simulink model "Chapter6"  (R2024b)
settings: Solver=ode4  StartTime=0.0  StopTime=SIM.StopTime  FixedStep=SIM.FixedStepSize  RelTol=1e-3
values from neighbouring files (symbols this model uses):
  AP = computeAutopilotGains(MAV, TRIM, TFS, DES)    [ch6_main.m]    (also in computeAutopilotGains.m = struct())
  CMD = struct()    [ch6_main.m]
  DES = loadDesignParams()    [ch6_main.m]    (also in loadDesignParams.m = struct())
  LIM = loadSafetyLimits()    [ch6_main.m]
  TRIM =     [ch6.mat]    (also in ch6_main.m = findTrim(TRIM_MODEL, Va_trim, R_trim, gamma_trim, TRIM_DATA_; findTrim.m = struct())
undefined symbols (not defined in the file or in its folder): drawAircraft, MAV, plotter, SIM
libraries: simulink x8, matrix_library x2
(part 1 of 2)
settings Model: Creator=emrec  LastModifiedBy=emrec

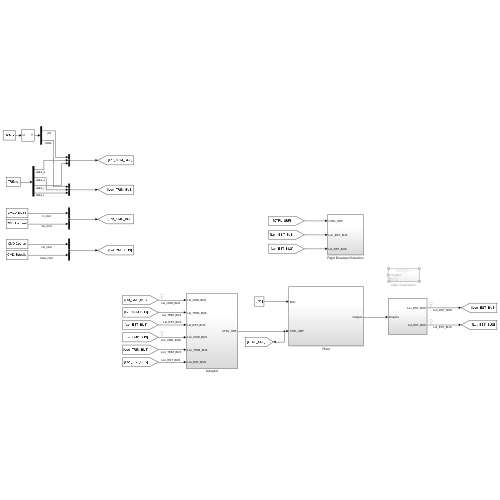
[thumbnail: Simulink's stored preview of the top-level diagram]
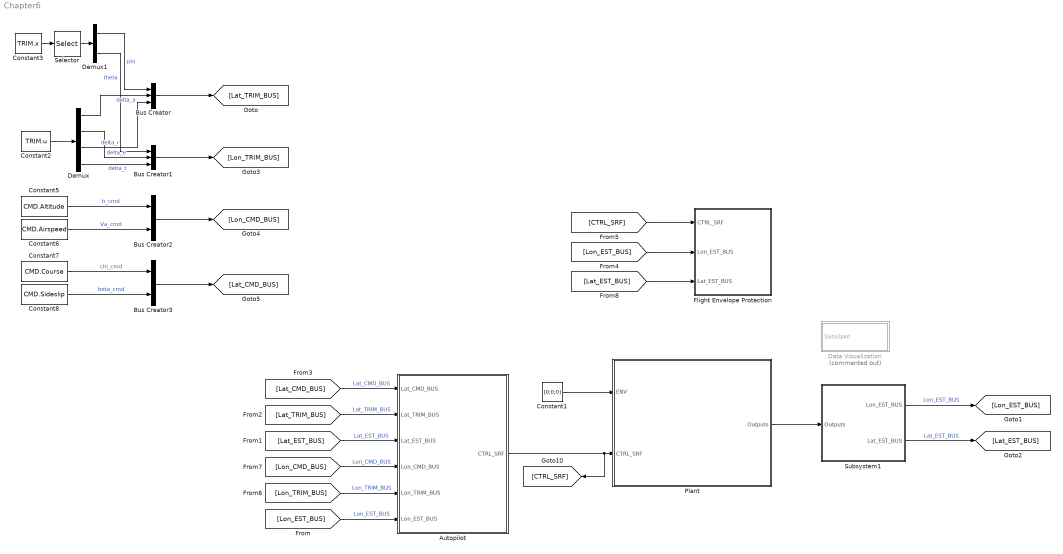
== system Chapter6 ==
  Autopilot : Subsystem
  Bus Creator : BusCreator  Inputs=3
  Bus Creator1 : BusCreator  Inputs=3
  Bus Creator2 : BusCreator  Inputs=2
  Bus Creator3 : BusCreator  Inputs=2
  Constant1 : Constant  Value=[0;0;0]
  Constant2 : Constant  Value=TRIM.u
  Constant3 : Constant  Value=TRIM.x
  Constant5 : Constant  Value=CMD.Altitude
  Constant6 : Constant  Value=CMD.Airspeed
  Constant7 : Constant  Value=CMD.Course
  Constant8 : Constant  Value=CMD.Sideslip
  Data Visualization : Subsystem  Commented=on  Variant=on
  Demux : Demux
  Demux1 : Demux  Outputs=2
  Flight Envelope Protection : Subsystem
  Plant : Subsystem
  Selector : Selector  InputPortWidth=12  IndexOptions=Index vector (dialog)  Indices=[7,8]  OutputSizes=1
  Subsystem1 : Subsystem
  wires:
  Constant1/1 -> Plant/1(ENV)
  Constant2/1 -> Demux/1
  Demux/1 -> Bus Creator/2  "delta_a"
  Demux/2 -> Bus Creator1/2  "delta_e"
  Demux/3 -> Bus Creator/3  "delta_r"
  Demux/4 -> Bus Creator1/3  "delta_t"
  Plant/1(Outputs) -> Subsystem1/1(Outputs)
  Subsystem1/1(Lon_EST_BUS) -> [Lon_EST_BUS]  "Lon_EST_BUS"
  Subsystem1/2(Lat_EST_BUS) -> [Lat_EST_BUS]  "Lat_EST_BUS"
  Bus Creator/1 -> [Lat_TRIM_BUS]
  Bus Creator1/1 -> [Lon_TRIM_BUS]
  Constant6/1 -> Bus Creator2/2  "Va_cmd"
  Constant5/1 -> Bus Creator2/1  "h_cmd"
  Bus Creator2/1 -> [Lon_CMD_BUS]
  Bus Creator3/1 -> [Lat_CMD_BUS]
  Constant7/1 -> Bus Creator3/1  "chi_cmd"
  Constant8/1 -> Bus Creator3/2  "beta_cmd"
  Constant3/1 -> Selector/1
  Selector/1 -> Demux1/1
  Demux1/1 -> Bus Creator/1  "phi"
  Demux1/2 -> Bus Creator1/1  "theta"
  Autopilot/1(CTRL_SRF) -> [CTRL_SRF], Plant/2(CTRL_SRF)
  [Lat_CMD_BUS] -> Autopilot/1(Lat_CMD_BUS)  "Lat_CMD_BUS"
  [Lat_TRIM_BUS] -> Autopilot/2(Lat_TRIM_BUS)  "Lat_TRIM_BUS"
  [Lat_EST_BUS] -> Autopilot/3(Lat_EST_BUS)  "Lat_EST_BUS"
  [Lon_CMD_BUS] -> Autopilot/4(Lon_CMD_BUS)  "Lon_CMD_BUS"
  [Lon_TRIM_BUS] -> Autopilot/5(Lon_TRIM_BUS)  "Lon_TRIM_BUS"
  [Lon_EST_BUS] -> Autopilot/6(Lon_EST_BUS)  "Lon_EST_BUS"
  [CTRL_SRF] -> Flight Envelope Protection/1(CTRL_SRF)
  [Lon_EST_BUS] -> Flight Envelope Protection/2(Lon_EST_BUS)
  [Lat_EST_BUS] -> Flight Envelope Protection/3(Lat_EST_BUS)

== system Chapter6/Autopilot ==
  Lat_CMD_BUS : Inport
  Lat_TRIM_BUS : Inport  Port=2
  Lat_EST_BUS : Inport  Port=3
  Lon_CMD_BUS : Inport  Port=4
  Lon_TRIM_BUS : Inport  Port=5
  Lon_EST_BUS : Inport  Port=6
  Lateral Autopilot : Subsystem
  Longitudinal Autopilot : Subsystem
  Mux1 : Mux
  CTRL_SRF : Outport
  wires:
  [delta_a] -> Mux1/1
  Lateral Autopilot/2(delta_r) -> [delta_r]
  [delta_t] -> Mux1/4
  Mux1/1 -> CTRL_SRF/1  "CTRL_SRF"
  Longitudinal Autopilot/1(delta_e) -> [delta_e]
  Longitudinal Autopilot/2(delta_t) -> [delta_t]
  [delta_e] -> Mux1/2
  Lon_CMD_BUS/1 -> Longitudinal Autopilot/1(Lon_CMD_BUS)
  [delta_r] -> Mux1/3
  Lateral Autopilot/1(delta_a) -> [delta_a]
  Lat_EST_BUS/1 -> Lateral Autopilot/3(Lat_EST_BUS)
  Lon_EST_BUS/1 -> Longitudinal Autopilot/3(Lon_EST_BUS)
  Lat_CMD_BUS/1 -> Lateral Autopilot/1(Lat_CMD_BUS)
  Lon_TRIM_BUS/1 -> Longitudinal Autopilot/2(Lon_TRIM_BUS)
  Lat_TRIM_BUS/1 -> Lateral Autopilot/2(Lat_TRIM_BUS)

== system Chapter6/Data Visualization ==
  note: 1) Add Subsystem or Model blocks as valid variant choices.
      | 2) You cannot connect blocks at this level. At simulation, connectivity is automatically
      | determined, based on the active variant and port name matching.
  Data2plot : Inport
  Data Storing : Subsystem  VariantControl=PLOTTING_MODEL == 2
  Online Plotting : Subsystem  VariantControl=PLOTTING_MODEL == 1

== system Chapter6/Flight Envelope Protection ==
  CTRL_SRF : Inport
  Lon_EST_BUS : Inport  Port=2
  Lat_EST_BUS : Inport  Port=3
  Abs : Abs  SaturateOnIntegerOverflow=off
  Bus Selector : BusSelector  OutputSignals=p_nh_hat,Va_hat,theta_hat
  Compare To Constant : simulink/Logic and Bit Operations/Compare To Constant  relop=<  const=LIM.Altitude.min  OutDataTypeStr=boolean
  Compare To Constant1 : simulink/Logic and Bit Operations/Compare To Constant  relop=>  const=LIM.Altitude.max  OutDataTypeStr=boolean
  Compare To Constant2 : simulink/Logic and Bit Operations/Compare To Constant  relop=>  const=LIM.Airspeed.max  OutDataTypeStr=boolean
  Compare To Constant3 : simulink/Logic and Bit Operations/Compare To Constant  relop=>  const=LIM.Pitch.max  OutDataTypeStr=boolean
  Logical Operator : Logic  Operator=OR  Inputs=4  AllPortsSameDT=off  OutDataTypeStr=boolean
  Selector : Selector  InputPortWidth=2  IndexOptions=Index vector (dialog)  Indices=[2]  OutputSizes=1
  Stop Simulation : Stop
  wires:
  Lon_EST_BUS/1 -> Bus Selector/1
  Bus Selector/1 -> Selector/1  "<p_nh_hat>"
  Selector/1 -> Compare To Constant/1, Compare To Constant1/1
  Compare To Constant/1 -> Logical Operator/1  "crash"
  Compare To Constant1/1 -> Logical Operator/2  "excess_h"
  Compare To Constant2/1 -> Logical Operator/3  "excess_Va"
  Bus Selector/3 -> Abs/1  "<theta_hat>"
  Abs/1 -> Compare To Constant3/1
  Bus Selector/2 -> Compare To Constant2/1  "<Va_hat>"
  Compare To Constant3/1 -> Logical Operator/4  "excess_theta"
  Logical Operator/1 -> Stop Simulation/1

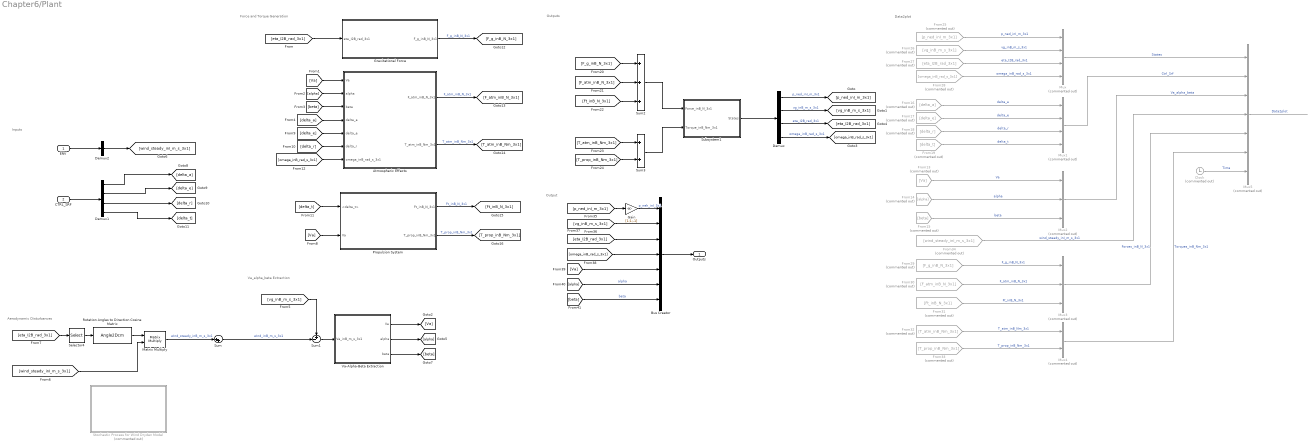
== system Chapter6/Plant ==
  note: Aerodynamic Disturbances
  note: Force and Torque Generation
  note: Inputs
  note: Outputs
  note: Data2plot
  note: Va_alpha_beta Extraction
  note: Output
  ENV : Inport
  CTRL_SRF : Inport  Port=2
  Atmospheric Effects : Subsystem
  Bus Creator : BusCreator  Inputs=7
  Clock : Clock  Commented=on
  Demux : Demux
  Demux1 : Demux
  Demux2 : Demux  Outputs=1
  From13 : From  Commented=on  GotoTag=Va
  From14 : From  Commented=on  GotoTag=alpha
  From15 : From  Commented=on  GotoTag=beta
  From16 : From  Commented=on  GotoTag=delta_a
  From17 : From  Commented=on  GotoTag=delta_e
  From18 : From  Commented=on  GotoTag=delta_r
  From19 : From  Commented=on  GotoTag=delta_t
  From25 : From  Commented=on  GotoTag=p_ned_inI_m_3x1
  From26 : From  Commented=on  GotoTag=vg_inB_m_s_3x1
  From27 : From  Commented=on  GotoTag=eta_I2B_rad_3x1
  From28 : From  Commented=on  GotoTag=omega_inB_rad_s_3x1
  From29 : From  Commented=on  GotoTag=F_g_inB_N_3x1
  From30 : From  Commented=on  GotoTag=F_atm_inB_N_3x1
  From31 : From  Commented=on  GotoTag=Ft_inB_N_3x1
  From32 : From  Commented=on  GotoTag=T_atm_inB_Nm_3x1
  From33 : From  Commented=on  GotoTag=T_prop_inB_Nm_3x1
  From34 : From  Commented=on  GotoTag=wind_steady_inI_m_s_3x1
  Gain : Gain  Gain=[1;1;-1]
  Gravitational Force : Subsystem
  Matrix Multiply : Product  Multiplication=Matrix(*)
  Mux : Mux  Commented=on
  Mux1 : Mux  Commented=on
  Mux2 : Mux  Commented=on  Inputs=3
  Mux3 : Mux  Commented=on  Inputs=3
  Mux4 : Mux  Commented=on  Inputs=2
  Mux5 : Mux  Commented=on  Inputs=7
  Propulsion System : Subsystem
  Rotation Angles to Direction Cosine Matrix : Angle2Dcm
      settings: AttributesFormatString=Rotation Order: %<rotationOrder>
  Selector4 : Selector  InputPortWidth=3  IndexOptions=Index vector (dialog)  Indices=[3 2 1]  OutputSizes=1
  Stochastic Process for Wind Dryden Model : Subsystem  Commented=on
  Subsystem1 : Subsystem  mask{init_states=MAV.init_states, J_B_B=MAV.J_B_B, m=MAV.m}
      mask prompts: init_states "Initial state values"; J_B_B "Inertia matrix (Kg.m3)"; m "Mass (Kg)"
  Sum : Sum  Inputs=|++
  Sum1 : Sum  Inputs=+-|
  Sum2 : Sum  Inputs=+++
  Sum3 : Sum
  Va-Alpha-Beta Extraction : Subsystem
  Outputs : Outport
  wires:
  Bus Creator/1 -> Outputs/1
  [omega_inB_rad_s_3x1] -> Bus Creator/4
  [eta_I2B_rad_3x1] -> Bus Creator/3
  [vg_inB_m_s_3x1] -> Bus Creator/2
  [p_ned_inI_m_3x1] -> Gain/1
  [Va] -> Propulsion System/2(Va)
  [delta_t] -> Propulsion System/1(<delta_t>)
  Propulsion System/1(Ft_inB_N_3x1) -> [Ft_inB_N_3x1]  "Ft_inB_N_3x1"
  Propulsion System/2(T_prop_inB_Nm_3x1) -> [T_prop_inB_Nm_3x1]  "T_prop_inB_Nm_3x1"
  Mux4/1 -> Mux5/6  "Torques_inB_Nm_3x1"
  Mux2/1 -> Mux5/3  "Va_alpha_beta"
  From34/1 -> Mux5/4  "wind_steady_inI_m_s_3x1"
  Clock/1 -> Mux5/7  "Time"
  Mux5/1 -> ?  "Data2plot"
  From33/1 -> Mux4/2  "T_prop_inB_Nm_3x1"
  From32/1 -> Mux4/1  "T_atm_inB_Nm_3x1"
  Mux3/1 -> Mux5/5  "Forces_inB_N_3x1"
  From29/1 -> Mux3/1  "F_g_inB_N_3x1"
  From30/1 -> Mux3/2  "F_atm_inB_N_3x1"
  From31/1 -> Mux3/3  "Ft_inB_N_3x1"
  From15/1 -> Mux2/3  "beta"
  From13/1 -> Mux2/1  "Va"
  From14/1 -> Mux2/2  "alpha"
  Mux1/1 -> Mux5/2  "Ctrl_Srf"
  From19/1 -> Mux1/4  "delta_t"
  From18/1 -> Mux1/3  "delta_r"
  From17/1 -> Mux1/2  "delta_e"
  From16/1 -> Mux1/1  "delta_a"
  Mux/1 -> Mux5/1  "States"
  From28/1 -> Mux/4  "omega_inB_rad_s_3x1"
  From27/1 -> Mux/3  "eta_I2B_rad_3x1"
  From26/1 -> Mux/2  "vg_inB_m_s_3x1"
  From25/1 -> Mux/1  "p_ned_inI_m_3x1"
  [T_prop_inB_Nm_3x1] -> Sum3/2
  [T_atm_inB_Nm_3x1] -> Sum3/1
  [Ft_inB_N_3x1] -> Sum2/3
  [F_atm_inB_N_3x1] -> Sum2/2
  [F_g_inB_N_3x1] -> Sum2/1
  Gravitational Force/1(F_g_inB_N_3x1) -> [F_g_inB_N_3x1]  "F_g_inB_N_3x1"
  Atmospheric Effects/1(F_atm_inB_N_3x1) -> [F_atm_inB_N_3x1]  "F_atm_inB_N_3x1"
  Atmospheric Effects/2(T_atm_inB_Nm_3x1) -> [T_atm_inB_Nm_3x1]  "T_atm_inB_Nm_3x1"
  Demux1/2 -> [delta_e]
  ENV/1 -> Demux2/1
  Sum1/1 -> Va-Alpha-Beta Extraction/1(Va_inB_m_s_3x1)
  [wind_steady_inI_m_s_3x1] -> Matrix Multiply/2
  Demux2/1 -> [wind_steady_inI_m_s_3x1]
  Selector4/1 -> Rotation Angles to Direction Cosine Matrix/1
  Demux1/4 -> [delta_t]
  [Va] -> Atmospheric Effects/1(Va)
  Va-Alpha-Beta Extraction/1(Va) -> [Va]
  Demux/4 -> [omega_inB_rad_s_3x1]  "omega_inB_rad_s_3x1"
  [delta_r] -> Atmospheric Effects/6(delta_r)
  [delta_a] -> Atmospheric Effects/4(delta_a)
  Matrix Multiply/1 -> Sum/1  "wind_steady_inB_m_s_3x1"
  [delta_e] -> Atmospheric Effects/5(delta_e)
  Subsystem1/1(States) -> Demux/1
  Va-Alpha-Beta Extraction/3(beta) -> [beta]
  Demux/1 -> [p_ned_inI_m_3x1]  "p_ned_inI_m_3x1"
  CTRL_SRF/1 -> Demux1/1
  Demux1/1 -> [delta_a]
  Demux/3 -> [eta_I2B_rad_3x1]  "eta_I2B_rad_3x1"
  Sum/1 -> Sum1/2  "wind_inB_m_s_3x1"
  [vg_inB_m_s_3x1] -> Sum1/1
  Demux/2 -> [vg_inB_m_s_3x1]  "vg_inB_m_s_3x1"
  [eta_I2B_rad_3x1] -> Selector4/1
  Rotation Angles to Direction Cosine Matrix/1 -> Matrix Multiply/1
  [eta_I2B_rad_3x1] -> Gravitational Force/1(eta_I2B_rad_3x1)
  Sum3/1 -> Subsystem1/2(Torque_inB_Nm_3x1)
  Va-Alpha-Beta Extraction/2(alpha) -> [alpha]
  Sum2/1 -> Subsystem1/1(Force_inB_N_3x1)
  [alpha] -> Atmospheric Effects/2(alpha)
  [beta] -> Atmospheric Effects/3(beta)
  Demux1/3 -> [delta_r]
  [omega_inB_rad_s_3x1] -> Atmospheric Effects/7(omega_inB_rad_s_3x1)
  [Va] -> Bus Creator/5
  [alpha] -> Bus Creator/6  "alpha"
  [beta] -> Bus Creator/7  "beta"
  Gain/1 -> Bus Creator/1  "p_neh_inI_3x1"

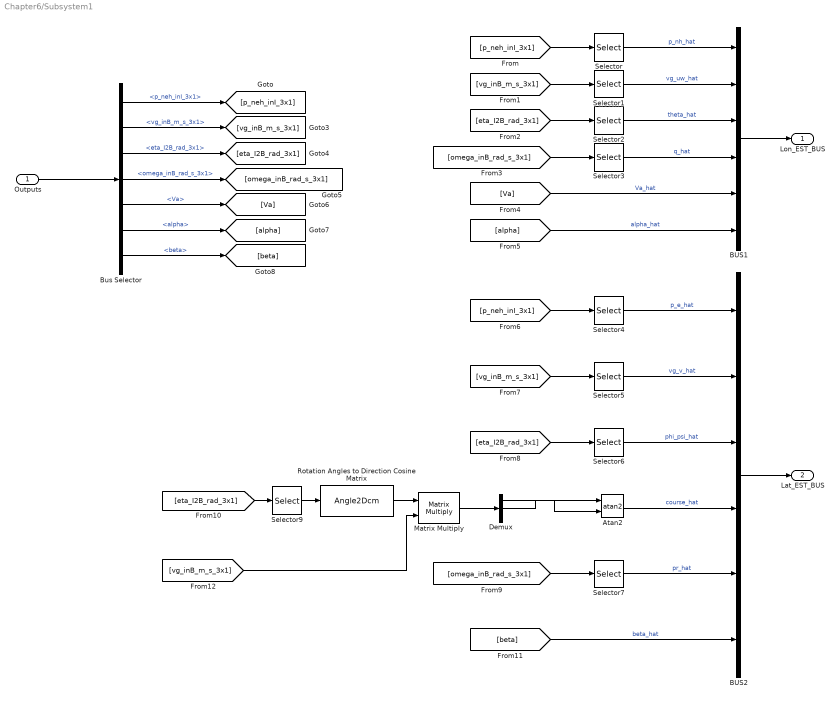
== system Chapter6/Subsystem1 ==
  Outputs : Inport
  Atan2 : Trigonometry  Operator=atan2
  BUS1 : BusCreator  Inputs=6
  BUS2 : BusCreator  Inputs=6
  Bus Selector : BusSelector  OutputSignals=p_neh_inI_3x1,vg_inB_m_s_3x1,eta_I2B_rad_3x1,omega_inB_rad_s_3x1,Va,alpha,beta
  Demux : Demux  Outputs=3
  Matrix Multiply : Product  Multiplication=Matrix(*)
  Rotation Angles to Direction Cosine Matrix : Angle2Dcm
      settings: AttributesFormatString=Rotation Order: %<rotationOrder>
  Selector : Selector  InputPortWidth=3  IndexOptions=Index vector (dialog)  Indices=[1 3]  OutputSizes=1
  Selector1 : Selector  InputPortWidth=3  IndexOptions=Index vector (dialog)  Indices=[1 3]  OutputSizes=1
  Selector{2..5} (4 alike) : Selector  InputPortWidth=3  IndexOptions=Index vector (dialog)  Indices=[2]  OutputSizes=1
  Selector6 : Selector  InputPortWidth=3  IndexOptions=Index vector (dialog)  Indices=[1,3]  OutputSizes=1
  Selector7 : Selector  InputPortWidth=3  IndexOptions=Index vector (dialog)  Indices=[1, 3]  OutputSizes=1
  Selector9 : Selector  InputPortWidth=3  IndexOptions=Index vector (dialog)  Indices=[3 2 1]  OutputSizes=1
  Lon_EST_BUS : Outport
  Lat_EST_BUS : Outport  Port=2
  wires:
  Outputs/1 -> Bus Selector/1
  BUS1/1 -> Lon_EST_BUS/1
  Bus Selector/1 -> [p_neh_inI_3x1]  "<p_neh_inI_3x1>"
  Bus Selector/2 -> [vg_inB_m_s_3x1]  "<vg_inB_m_s_3x1>"
  Bus Selector/3 -> [eta_I2B_rad_3x1]  "<eta_I2B_rad_3x1>"
  Bus Selector/4 -> [omega_inB_rad_s_3x1]  "<omega_inB_rad_s_3x1>"
  Bus Selector/5 -> [Va]  "<Va>"
  Bus Selector/6 -> [alpha]  "<alpha>"
  Bus Selector/7 -> [beta]  "<beta>"
  [p_neh_inI_3x1] -> Selector/1
  Selector/1 -> BUS1/1  "p_nh_hat"
  [vg_inB_m_s_3x1] -> Selector1/1
  Selector1/1 -> BUS1/2  "vg_uw_hat"
  [eta_I2B_rad_3x1] -> Selector2/1
  Selector2/1 -> BUS1/3  "theta_hat"
  [omega_inB_rad_s_3x1] -> Selector3/1
  Selector3/1 -> BUS1/4  "q_hat"
  [Va] -> BUS1/5  "Va_hat"
  [alpha] -> BUS1/6  "alpha_hat"
  [beta] -> BUS2/6  "beta_hat"
  Selector7/1 -> BUS2/5  "pr_hat"
  [omega_inB_rad_s_3x1] -> Selector7/1
  Selector6/1 -> BUS2/3  "phi_psi_hat"
  [eta_I2B_rad_3x1] -> Selector6/1
  Selector5/1 -> BUS2/2  "vg_v_hat"
  [vg_inB_m_s_3x1] -> Selector5/1
  Selector4/1 -> BUS2/1  "p_e_hat"
  [p_neh_inI_3x1] -> Selector4/1
  BUS2/1 -> Lat_EST_BUS/1
  Atan2/1 -> BUS2/4  "course_hat"
  [vg_inB_m_s_3x1] -> Matrix Multiply/2
  Selector9/1 -> Rotation Angles to Direction Cosine Matrix/1
  Rotation Angles to Direction Cosine Matrix/1 -> Matrix Multiply/1
  [eta_I2B_rad_3x1] -> Selector9/1
  Matrix Multiply/1 -> Demux/1
  Demux/2 -> Atan2/1
  Demux/1 -> Atan2/2

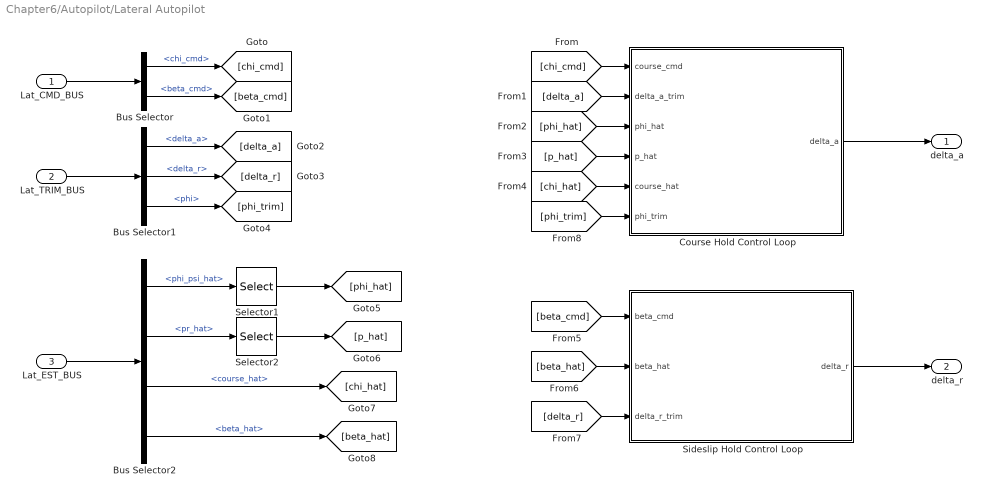
== system Chapter6/Autopilot/Lateral Autopilot ==
  Lat_CMD_BUS : Inport
  Lat_TRIM_BUS : Inport  Port=2
  Lat_EST_BUS : Inport  Port=3
  Bus Selector : BusSelector  OutputSignals=chi_cmd,beta_cmd
  Bus Selector1 : BusSelector  OutputSignals=delta_a,delta_r,phi
  Bus Selector2 : BusSelector  OutputSignals=phi_psi_hat,pr_hat,course_hat,beta_hat
  Course Hold Control Loop : Subsystem
  Selector1 : Selector  InputPortWidth=2  IndexOptions=Index vector (dialog)  Indices=1  OutputSizes=1
  Selector2 : Selector  InputPortWidth=2  IndexOptions=Index vector (dialog)  Indices=1  OutputSizes=1
  Sideslip Hold Control Loop : Subsystem
  delta_a : Outport
  delta_r : Outport  Port=2
  wires:
  Sideslip Hold Control Loop/1(delta_r) -> delta_r/1
  Course Hold Control Loop/1(delta_a) -> delta_a/1
  Lat_CMD_BUS/1 -> Bus Selector/1
  Bus Selector/1 -> [chi_cmd]  "<chi_cmd>"
  Bus Selector/2 -> [beta_cmd]  "<beta_cmd>"
  Lat_TRIM_BUS/1 -> Bus Selector1/1
  Bus Selector1/1 -> [delta_a]  "<delta_a>"
  Bus Selector1/2 -> [delta_r]  "<delta_r>"
  Lat_EST_BUS/1 -> Bus Selector2/1
  Selector1/1 -> [phi_hat]
  Bus Selector2/2 -> Selector2/1  "<pr_hat>"
  Bus Selector2/1 -> Selector1/1  "<phi_psi_hat>"
  Selector2/1 -> [p_hat]
  Bus Selector2/3 -> [chi_hat]  "<course_hat>"
  Bus Selector2/4 -> [beta_hat]  "<beta_hat>"
  [chi_cmd] -> Course Hold Control Loop/1(course_cmd)
  [delta_a] -> Course Hold Control Loop/2(delta_a_trim)
  [phi_hat] -> Course Hold Control Loop/3(phi_hat)
  [p_hat] -> Course Hold Control Loop/4(p_hat)
  [chi_hat] -> Course Hold Control Loop/5(course_hat)
  [beta_cmd] -> Sideslip Hold Control Loop/1(beta_cmd)
  [beta_hat] -> Sideslip Hold Control Loop/2(beta_hat)
  [delta_r] -> Sideslip Hold Control Loop/3(delta_r_trim)
  Bus Selector1/3 -> [phi_trim]  "<phi>"
  [phi_trim] -> Course Hold Control Loop/6(phi_trim)

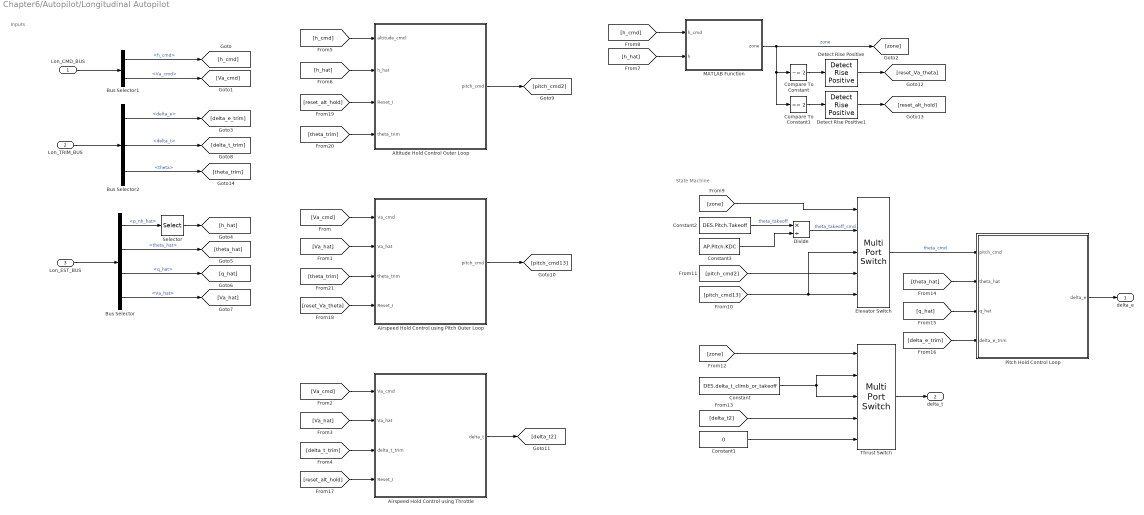
== system Chapter6/Autopilot/Longitudinal Autopilot ==
  note: Inputs
  note: State Machine
  Lon_CMD_BUS : Inport
  Lon_TRIM_BUS : Inport  Port=2
  Lon_EST_BUS : Inport  Port=3
  Airspeed Hold Control using Pitch Outer Loop : Subsystem
  "Airspeed Hold Control using Throttle " : Subsystem
  Altitude Hold Control Outer Loop : Subsystem
  Bus Selector : BusSelector  OutputSignals=p_nh_hat,theta_hat,q_hat,Va_hat
  Bus Selector1 : BusSelector  OutputSignals=h_cmd,Va_cmd
  Bus Selector2 : BusSelector  OutputSignals=delta_e,delta_t,theta
  Compare To Constant : simulink/Logic and Bit Operations/Compare To Constant  relop=~=  const=2  OutDataTypeStr=boolean
  Compare To Constant1 : simulink/Logic and Bit Operations/Compare To Constant  relop===  const=2  OutDataTypeStr=boolean
  Constant : Constant  Value=DES.delta_t_climb_or_takeoff
  Constant1 : Constant  Value=0
  Constant2 : Constant  Value=DES.Pitch.Takeoff
  Constant3 : Constant  Value=AP.Pitch.KDC
  Detect Rise Positive : simulink/Logic and Bit Operations/Detect Rise Positive  vinit=0  OutDataTypeStr=boolean
  Detect Rise Positive1 : simulink/Logic and Bit Operations/Detect Rise Positive  vinit=0  OutDataTypeStr=boolean
  Divide : Product  Inputs=*/
  Elevator Switch : MultiPortSwitch  DataPortOrder=Zero-based contiguous  Inputs=4  zeroidx=on  SaturateOnIntegerOverflow=off  InputSameDT=off
  MATLAB Function : MATLAB Function  TreatAsAtomicUnit=on  SystemSampleTime=SIM.FixedStepSize
  Pitch Hold Control Loop : Subsystem
  Selector : Selector  InputPortWidth=2  IndexOptions=Index vector (dialog)  Indices=2  OutputSizes=1
  Thrust Switch : MultiPortSwitch  DataPortOrder=Zero-based contiguous  Inputs=4  zeroidx=on  SaturateOnIntegerOverflow=off  InputSameDT=off
  delta_e : Outport
  delta_t : Outport  Port=2
  wires:
  Pitch Hold Control Loop/1(delta_e) -> delta_e/1
  [h_hat] -> MATLAB Function/2(h)
  Constant/1 -> Thrust Switch/2, Thrust Switch/3
  Constant1/1 -> Thrust Switch/5
  Thrust Switch/1 -> delta_t/1
  Constant2/1 -> Divide/1  "theta_takeoff"
  Constant3/1 -> Divide/2
  Divide/1 -> Elevator Switch/2  "theta_takeoff_cmd"
  [Va_cmd] -> Airspeed Hold Control using Pitch Outer Loop/1(Va_cmd)
  [Va_hat] -> Airspeed Hold Control using Pitch Outer Loop/2(Va_hat)
  Lon_EST_BUS/1 -> Bus Selector/1
  Bus Selector/1 -> Selector/1  "<p_nh_hat>"
  Selector/1 -> [h_hat]
  Bus Selector/2 -> [theta_hat]  "<theta_hat>"
  Bus Selector/3 -> [q_hat]  "<q_hat>"
  Bus Selector/4 -> [Va_hat]  "<Va_hat>"
  Lon_CMD_BUS/1 -> Bus Selector1/1
  Bus Selector1/1 -> [h_cmd]  "<h_cmd>"
  Bus Selector1/2 -> [Va_cmd]  "<Va_cmd>"
  Bus Selector2/1 -> [delta_e_trim]  "<delta_e>"
  Lon_TRIM_BUS/1 -> Bus Selector2/1
  Bus Selector2/2 -> [delta_t_trim]  "<delta_t>"
  [Va_cmd] -> "Airspeed Hold Control using Throttle "/1(Va_cmd)
  [Va_hat] -> "Airspeed Hold Control using Throttle "/2(Va_hat)
  [delta_t_trim] -> "Airspeed Hold Control using Throttle "/3(delta_t_trim)
  [h_cmd] -> Altitude Hold Control Outer Loop/1(altitude_cmd)
  [h_hat] -> Altitude Hold Control Outer Loop/2(h_hat)
  Altitude Hold Control Outer Loop/1(pitch_cmd) -> [pitch_cmd2]
  Airspeed Hold Control using Pitch Outer Loop/1(pitch_cmd) -> [pitch_cmd13]
  "Airspeed Hold Control using Throttle "/1(delta_t) -> [delta_t2]
  [h_cmd] -> MATLAB Function/1(h_cmd)
  [zone] -> Elevator Switch/1
  [pitch_cmd13] -> Elevator Switch/5, Elevator Switch/3
  [pitch_cmd2] -> Elevator Switch/4
  [zone] -> Thrust Switch/1
  [delta_t2] -> Thrust Switch/4
  [theta_hat] -> Pitch Hold Control Loop/2(theta_hat)
  [q_hat] -> Pitch Hold Control Loop/3(q_hat)
  [delta_e_trim] -> Pitch Hold Control Loop/4(delta_e_trim)
  Compare To Constant/1 -> Detect Rise Positive/1
  Compare To Constant1/1 -> Detect Rise Positive1/1
  Detect Rise Positive/1 -> [reset_Va_theta]
  Detect Rise Positive1/1 -> [reset_alt_hold]
  [reset_alt_hold] -> "Airspeed Hold Control using Throttle "/4(Reset_I)
  [reset_Va_theta] -> Airspeed Hold Control using Pitch Outer Loop/4(Reset_I)
  [reset_alt_hold] -> Altitude Hold Control Outer Loop/3(Reset_I)
  Bus Selector2/3 -> [theta_trim]  "<theta>"
  [theta_trim] -> Altitude Hold Control Outer Loop/4(theta_trim)
  [theta_trim] -> Airspeed Hold Control using Pitch Outer Loop/3(theta_trim)
  MATLAB Function/1(zone) -> [zone], Compare To Constant1/1, Compare To Constant/1  "zone"
  Elevator Switch/1 -> Pitch Hold Control Loop/1(pitch_cmd)  "theta_cmd"

== system Chapter6/Data Visualization/Data Storing ==
  Data2plot : Inport
  To Workspace : ToWorkspace  VariableName=simout  SampleTime=-1
  wires:
  Data2plot/1 -> To Workspace/1

== system Chapter6/Data Visualization/Online Plotting ==
  Data2plot : Inport
  Aircraft Body Animation : MATLABFcn  MATLABFcn=drawAircraft(u)  OutputDimensions=0
  Clock : Clock
  Mux : Mux  Inputs=2
  Plot Graphs : MATLABFcn  MATLABFcn=plotter(u)  OutputDimensions=0
  Selector : Selector  InputPortWidth=38  IndexOptions=Index vector (dialog)  Indices=[1:12]  OutputSizes=1
  wires:
  Mux/1 -> Aircraft Body Animation/1
  Clock/1 -> Mux/2
  Selector/1 -> Mux/1
  Data2plot/1 -> Plot Graphs/1, Selector/1

== system Chapter6/Plant/Atmospheric Effects ==
  Va : Inport
  alpha : Inport  Port=2
  beta : Inport  Port=3
  delta_a : Inport  Port=4
  delta_e : Inport  Port=5
  delta_r : Inport  Port=6
  omega_inB_rad_s_3x1 : Inport  Port=7
  Aerodynamic Effect on Latitude Motion : Subsystem
  Aerodynamic Effect on Longitudinal Motion : Subsystem
  Mux1 : Mux  Inputs=2
  Selector : Selector  InputPortWidth=3  IndexOptions=Index vector (dialog)  Indices=[2]  OutputSizes=1
  Selector1 : Selector  InputPortWidth=3  IndexOptions=Index vector (dialog)  Indices=[1 3]  OutputSizes=1
  Selector2 : Selector  InputPortWidth=6  IndexOptions=Index vector (dialog)  Indices=[1 4 2]  OutputSizes=1
  Selector3 : Selector  InputPortWidth=6  IndexOptions=Index vector (dialog)  Indices=[5 3 6]  OutputSizes=1
  F_atm_inB_N_3x1 : Outport
  T_atm_inB_Nm_3x1 : Outport  Port=2
  wires:
  Mux1/1 -> Selector3/1, Selector2/1
  Selector2/1 -> F_atm_inB_N_3x1/1  "F_atm_inB_N_3x1"
  delta_e/1 -> Aerodynamic Effect on Longitudinal Motion/1(delta_e)
  delta_a/1 -> Aerodynamic Effect on Latitude Motion/1(delta_a)
  Aerodynamic Effect on Longitudinal Motion/1(Fx_Fz_Tq_inB) -> Mux1/1
  alpha/1 -> Aerodynamic Effect on Longitudinal Motion/3(alpha)
  Aerodynamic Effect on Latitude Motion/1(Fy_Tp_Tr_inB) -> Mux1/2
  delta_r/1 -> Aerodynamic Effect on Latitude Motion/2(delta_r)
  omega_inB_rad_s_3x1/1 -> Selector1/1, Selector/1
  Va/1 -> Aerodynamic Effect on Latitude Motion/5(Va), Aerodynamic Effect on Longitudinal Motion/4(Va)
  beta/1 -> Aerodynamic Effect on Latitude Motion/3(beta)
  Selector3/1 -> T_atm_inB_Nm_3x1/1  "T_atm_inB_Nm_3x1"
  Selector/1 -> Aerodynamic Effect on Longitudinal Motion/2(q)
  Selector1/1 -> Aerodynamic Effect on Latitude Motion/4(p_r)

== system Chapter6/Plant/Gravitational Force ==
  eta_I2B_rad_3x1 : Inport
  Constant : Constant  Value=MAV.m * MAV.g
  Product : Product
  R_B_I_c3 : MATLAB Function  TreatAsAtomicUnit=on
  F_g_inB_N_3x1 : Outport
  wires:
  eta_I2B_rad_3x1/1 -> R_B_I_c3/1(u)
  R_B_I_c3/1(y) -> Product/1
  Constant/1 -> Product/2  "F_g_inI_N_3x1"
  Product/1 -> F_g_inB_N_3x1/1  "F_g_inB_N_3x1"

== system Chapter6/Plant/Propulsion System ==
  <delta_t> : Inport
  Va : Inport  Port=2
  Gain2 : Gain  Gain=MAV.K_motor
  Gain3 : Gain  Gain=MAV.S_prop * MAV.C_prop * MAV.rho/ 2
  Gain4 : Gain  Gain=-MAV.K_t_prop
  Gain5 : Gain  Gain=MAV.K_omega
  Square1 : Math  Operator=square
  Square2 : Math  Operator=square
  Square3 : Math  Operator=square
  Sum2 : Sum  Inputs=|+-
  vectorize_e1 : Gain  Gain=[1;0;0]
  vectorize_e2 : Gain  Gain=[1;0;0]
  Ft_inB_N_3x1 : Outport
  T_prop_inB_Nm_3x1 : Outport  Port=2
  wires:
  Gain5/1 -> Square3/1  "V_exit"
  Square3/1 -> Gain4/1
  vectorize_e2/1 -> T_prop_inB_Nm_3x1/1  "T_prop_inB_Nm_3x1"
  Va/1 -> Square2/1
  <delta_t>/1 -> Gain5/1, Gain2/1
  Gain3/1 -> Ft_inB_N_3x1/1  "Ft_inB_N_3x1"
  vectorize_e1/1 -> Gain3/1
  Square2/1 -> Sum2/2
  Sum2/1 -> vectorize_e1/1
  Gain4/1 -> vectorize_e2/1
  Square1/1 -> Sum2/1
  Gain2/1 -> Square1/1  "V_exit"

== system Chapter6/Plant/Stochastic Process for Wind Dryden Model ==

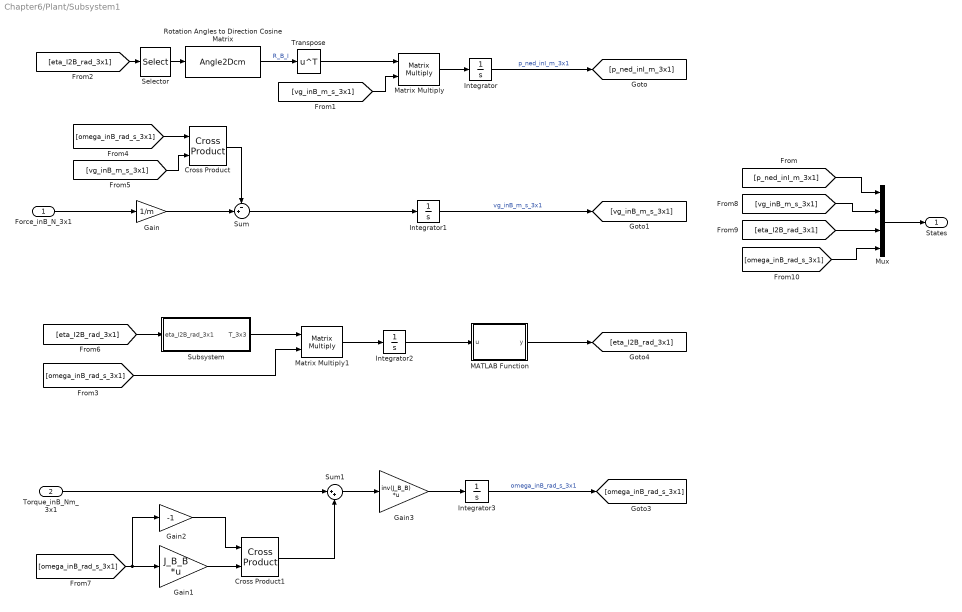
== system Chapter6/Plant/Subsystem1 ==
  Force_inB_N_3x1 : Inport
  Torque_inB_Nm_3x1 : Inport  Port=2
  Cross Product : matrix_library/Cross Product
  Cross Product1 : matrix_library/Cross Product
  Gain : Gain  Gain=1/m
  Gain1 : Gain  Gain=J_B_B  Multiplication=Matrix(K*u)
  Gain2 : Gain  Gain=-1
  Gain3 : Gain  Gain=inv(J_B_B)  Multiplication=Matrix(K*u)
  Integrator : Integrator  InitialCondition=init_states(1:3)
  Integrator1 : Integrator  InitialCondition=init_states(4:6)
  Integrator2 : Integrator  InitialCondition=init_states(7:9)
  Integrator3 : Integrator  InitialCondition=init_states(10:12)
  MATLAB Function : MATLAB Function  TreatAsAtomicUnit=on
  Matrix Multiply : Product  Multiplication=Matrix(*)
  Matrix Multiply1 : Product  Multiplication=Matrix(*)
  Mux : Mux
  Rotation Angles to Direction Cosine Matrix : Angle2Dcm
      settings: AttributesFormatString=Rotation Order: %<rotationOrder>
  Selector : Selector  InputPortWidth=3  IndexOptions=Index vector (dialog)  Indices=[3;2;1]  OutputSizes=1
  Subsystem : Subsystem
  Sum : Sum  Inputs=-+|
  Sum1 : Sum  Inputs=|++
  Transpose : Math  Operator=transpose
  States : Outport
  wires:
  MATLAB Function/1(y) -> [eta_I2B_rad_3x1]
  Gain3/1 -> Integrator3/1
  [p_ned_inI_m_3x1] -> Mux/1
  [omega_inB_rad_s_3x1] -> Cross Product/1
  Matrix Multiply1/1 -> Integrator2/1
  Gain1/1 -> Cross Product1/2
  [eta_I2B_rad_3x1] -> Subsystem/1(eta_I2B_rad_3x1)
  [omega_inB_rad_s_3x1] -> Matrix Multiply1/2
  Integrator1/1 -> [vg_inB_m_s_3x1]  "vg_inB_m_s_3x1"
  [vg_inB_m_s_3x1] -> Cross Product/2
  Selector/1 -> Rotation Angles to Direction Cosine Matrix/1
  [eta_I2B_rad_3x1] -> Selector/1
  Cross Product/1 -> Sum/1
  Integrator/1 -> [p_ned_inI_m_3x1]  "p_ned_inI_m_3x1"
  Matrix Multiply/1 -> Integrator/1
  Force_inB_N_3x1/1 -> Gain/1
  Rotation Angles to Direction Cosine Matrix/1 -> Transpose/1  "R_B_I"
  [omega_inB_rad_s_3x1] -> Gain2/1, Gain1/1
  Mux/1 -> States/1
  [omega_inB_rad_s_3x1] -> Mux/4
  Transpose/1 -> Matrix Multiply/1
  Integrator3/1 -> [omega_inB_rad_s_3x1]  "omega_inB_rad_s_3x1"
  [vg_inB_m_s_3x1] -> Matrix Multiply/2
  [eta_I2B_rad_3x1] -> Mux/3
  Torque_inB_Nm_3x1/1 -> Sum1/1
  Gain2/1 -> Cross Product1/1
  Sum1/1 -> Gain3/1
  Integrator2/1 -> MATLAB Function/1(u)
  [vg_inB_m_s_3x1] -> Mux/2
  Subsystem/1(T_3x3) -> Matrix Multiply1/1
  Cross Product1/1 -> Sum1/2
  Sum/1 -> Integrator1/1
  Gain/1 -> Sum/2

== system Chapter6/Plant/Va-Alpha-Beta Extraction ==
  note: To avoid zero division problem.
      | This logic and threshold is recommended by gemini.
  note: Va >= ||vr|| -> Va = 0 -> vr = 0
  Va_inB_m_s_3x1 : Inport
  Asin : Trigonometry  Operator=asin
  Constant : Constant
  Demux : Demux  Outputs=3
  Divide1 : Product  Inputs=*/
  Switch : Switch  Criteria=u2 > Threshold  SaturateOnIntegerOverflow=off  InputSameDT=off
  Trigonometric Function : Trigonometry  Operator=atan2  OutputSignalType=real
  norm2 : Subsystem
  Va : Outport
  alpha : Outport  Port=2
  beta : Outport  Port=3
  wires:
  Va_inB_m_s_3x1/1 -> norm2/1(Va_inB_m_s_3x1), Demux/1
  Demux/1 -> Trigonometric Function/2  "ur"
  Demux/2 -> Divide1/1  "vr"
  Demux/3 -> Trigonometric Function/1  "wr"
  norm2/1(Va) -> Switch/2, Switch/1, Va/1  "Va"
  Divide1/1 -> Asin/1
  Asin/1 -> beta/1
  Trigonometric Function/1 -> alpha/1
  Constant/1 -> Switch/3
  Switch/1 -> Divide1/2

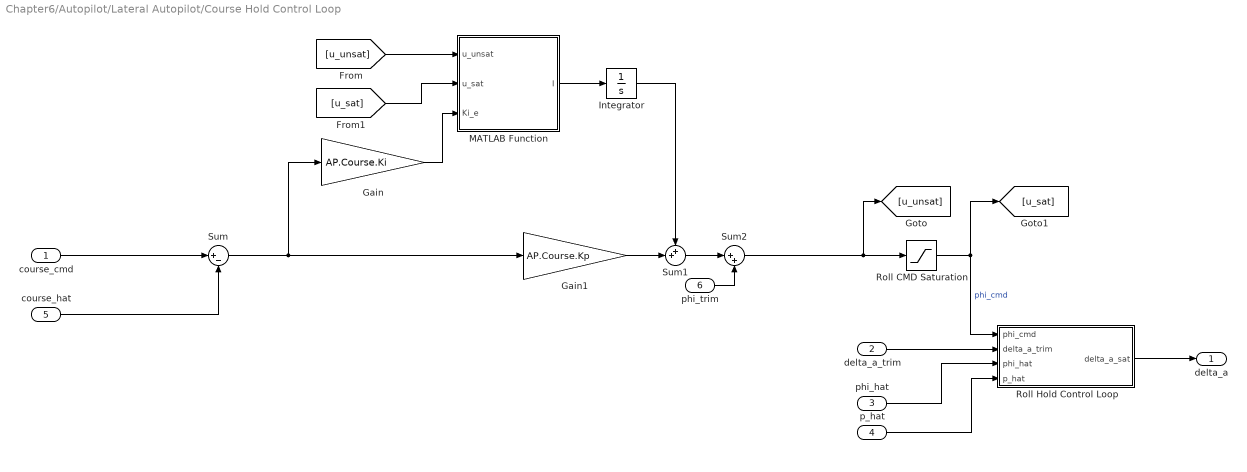
== system Chapter6/Autopilot/Lateral Autopilot/Course Hold Control Loop ==
  course_cmd : Inport
  delta_a_trim : Inport  Port=2
  phi_hat : Inport  Port=3
  p_hat : Inport  Port=4
  course_hat : Inport  Port=5
  phi_trim : Inport  Port=6
  Gain : Gain  Gain=AP.Course.Ki
  Gain1 : Gain  Gain=AP.Course.Kp
  Integrator : Integrator
  MATLAB Function : MATLAB Function  TreatAsAtomicUnit=on
  "Roll CMD Saturation " : Saturate  UpperLimit=DES.Roll.max  LowerLimit=-DES.Roll.max
  Roll Hold Control Loop : Subsystem
  Sum : Sum  Inputs=|+-
  Sum1 : Sum  Inputs=++|
  Sum2 : Sum  Inputs=|++
  delta_a : Outport
  wires:
  p_hat/1 -> Roll Hold Control Loop/4(p_hat)
  Integrator/1 -> Sum1/1
  Sum/1 -> Gain1/1, Gain/1
  Gain1/1 -> Sum1/2
  phi_hat/1 -> Roll Hold Control Loop/3(phi_hat)
  course_cmd/1 -> Sum/1
  course_hat/1 -> Sum/2
  delta_a_trim/1 -> Roll Hold Control Loop/2(delta_a_trim)
  Roll Hold Control Loop/1(delta_a_sat) -> delta_a/1
  Sum2/1 -> [u_unsat], "Roll CMD Saturation "/1
  "Roll CMD Saturation "/1 -> Roll Hold Control Loop/1(phi_cmd), [u_sat]  "phi_cmd"
  Gain/1 -> MATLAB Function/3(Ki_e)
  [u_unsat] -> MATLAB Function/1(u_unsat)
  [u_sat] -> MATLAB Function/2(u_sat)
  MATLAB Function/1(I) -> Integrator/1
  Sum1/1 -> Sum2/1
  phi_trim/1 -> Sum2/2

== system Chapter6/Autopilot/Lateral Autopilot/Sideslip Hold Control Loop ==
  beta_cmd : Inport
  beta_hat : Inport  Port=2
  delta_r_trim : Inport  Port=3
  Gain : Gain  Gain=-AP.Sideslip.Ki
  Gain1 : Gain  Gain=-AP.Sideslip.Kp
  MATLAB Function : MATLAB Function  TreatAsAtomicUnit=on
  Rudder Saturation : Saturate  UpperLimit=DES.delta_r_max  LowerLimit=-DES.delta_r_max
  Sideslip Hold I Action : Integrator
  Sum : Sum  Inputs=|+-
  Sum1 : Sum  Inputs=++|
  Sum2 : Sum  Inputs=|++
  delta_r : Outport
  wires:
  beta_cmd/1 -> Sum/1
  delta_r_trim/1 -> Sum2/2
  Sum1/1 -> Sum2/1  "Ddelta_r"
  Sum/1 -> Gain1/1, Gain/1
  Sum2/1 -> [u_unsat], Rudder Saturation/1
  Gain1/1 -> Sum1/2
  Rudder Saturation/1 -> [u_sat], delta_r/1  "delta_r_sat"
  beta_hat/1 -> Sum/2
  Sideslip Hold I Action/1 -> Sum1/1
  Gain/1 -> MATLAB Function/3(Ki_e)
  MATLAB Function/1(I) -> Sideslip Hold I Action/1
  [u_unsat] -> MATLAB Function/1(u_unsat)
  [u_sat] -> MATLAB Function/2(u_sat)

== system Chapter6/Autopilot/Longitudinal Autopilot/Airspeed Hold Control using Pitch Outer Loop ==
  Va_cmd : Inport
  Va_hat : Inport  Port=2
  theta_trim : Inport  Port=3
  Reset_I : Inport  Port=4
  Airspeed Hold using Pitch I Action : Integrator  ExternalReset=rising
  Gain1 : Gain  Gain=AP.Airspeed.Pitch.Kp
  Gain2 : Gain  Gain=AP.Airspeed.Pitch.Ki
  MATLAB Function : MATLAB Function  TreatAsAtomicUnit=on
  Pitch CMD Saturation : Saturate  UpperLimit=DES.Airspeed.Pitch.max  LowerLimit=-DES.Airspeed.Pitch.max
  Sum : Sum  Inputs=|+-
  Sum1 : Sum  Inputs=++|
  Sum2 : Sum  Inputs=|++
  pitch_cmd : Outport
  wires:
  Va_cmd/1 -> Sum/1
  Pitch CMD Saturation/1 -> pitch_cmd/1, [u_sat]  "pitch_cmd"
  Sum/1 -> Gain1/1, Gain2/1
  [u_unsat] -> MATLAB Function/1(u_unsat)
  MATLAB Function/1(I) -> Airspeed Hold using Pitch I Action/1
  [u_sat] -> MATLAB Function/2(u_sat)
  Gain1/1 -> Sum1/2
  Gain2/1 -> MATLAB Function/3(Ki_e)
  Airspeed Hold using Pitch I Action/1 -> Sum1/1
  Va_hat/1 -> Sum/2
  Reset_I/1 -> Airspeed Hold using Pitch I Action/2
  theta_trim/1 -> Sum2/2
  Sum1/1 -> Sum2/1  "Dtheta"
  Sum2/1 -> [u_unsat], Pitch CMD Saturation/1

== system Chapter6/Autopilot/Longitudinal Autopilot/Airspeed Hold Control using Throttle  ==
  Va_cmd : Inport
  Va_hat : Inport  Port=2
  delta_t_trim : Inport  Port=3
  Reset_I : Inport  Port=4
  Airspeed Hold using Throttle I Action : Integrator  ExternalReset=rising
  Gain1 : Gain  Gain=AP.Airspeed.Throttle.Kp
  Gain2 : Gain  Gain=AP.Airspeed.Throttle.Ki
  MATLAB Function : MATLAB Function  TreatAsAtomicUnit=on
  Sum : Sum  Inputs=|+-
  Sum1 : Sum  Inputs=++|
  Sum2 : Sum  Inputs=|++
  Throttle Saturation : Saturate  UpperLimit=DES.delta_t_max  LowerLimit=0
  delta_t : Outport
  wires:
  Va_hat/1 -> Sum/2
  Airspeed Hold using Throttle I Action/1 -> Sum1/1
  Gain2/1 -> MATLAB Function/3(Ki_e)
  Gain1/1 -> Sum1/2
  [u_sat] -> MATLAB Function/2(u_sat)
  MATLAB Function/1(I) -> Airspeed Hold using Throttle I Action/1
  [u_unsat] -> MATLAB Function/1(u_unsat)
  Sum/1 -> Gain2/1, Gain1/1
  Throttle Saturation/1 -> delta_t/1, [u_sat]
  Va_cmd/1 -> Sum/1
  Reset_I/1 -> Airspeed Hold using Throttle I Action/2
  Sum1/1 -> Sum2/1  "Ddelta_t"
  delta_t_trim/1 -> Sum2/2
  Sum2/1 -> [u_unsat], Throttle Saturation/1

== system Chapter6/Autopilot/Longitudinal Autopilot/Altitude Hold Control Outer Loop ==
  altitude_cmd : Inport
  h_hat : Inport  Port=2
  Reset_I : Inport  Port=3
  theta_trim : Inport  Port=4
  Altitude Hold I Action : Integrator  ExternalReset=rising
  Gain1 : Gain  Gain=AP.Altitude.Kp
  Gain2 : Gain  Gain=AP.Altitude.Ki
  MATLAB Function : MATLAB Function  TreatAsAtomicUnit=on
  Pitch CMD Saturation : Saturate  UpperLimit=DES.Altitude.Pitch.max  LowerLimit=-DES.Altitude.Pitch.max
  Sum : Sum  Inputs=|+-
  Sum1 : Sum  Inputs=++|
  Sum2 : Sum  Inputs=|++
  WrapToPi : Subsystem  Commented=through
  pitch_cmd : Outport
  wires:
  Sum/1 -> Gain2/1, Gain1/1
  WrapToPi/1(Out1) -> [u_unsat], Pitch CMD Saturation/1
  Gain2/1 -> MATLAB Function/3(Ki_e)
  Gain1/1 -> Sum1/2
  [u_sat] -> MATLAB Function/2(u_sat)
  Pitch CMD Saturation/1 -> [u_sat], pitch_cmd/1
  [u_unsat] -> MATLAB Function/1(u_unsat)
  altitude_cmd/1 -> Sum/1
  h_hat/1 -> Sum/2
  MATLAB Function/1(I) -> Altitude Hold I Action/1
  Altitude Hold I Action/1 -> Sum1/1
  Reset_I/1 -> Altitude Hold I Action/2
  Sum1/1 -> Sum2/1
  Sum2/1 -> WrapToPi/1(In1)
  theta_trim/1 -> Sum2/2

== system Chapter6/Autopilot/Longitudinal Autopilot/Pitch Hold Control Loop ==
  pitch_cmd : Inport
  theta_hat : Inport  Port=2
  q_hat : Inport  Port=3
  delta_e_trim : Inport  Port=4
  Elevator Saturation : Saturate  UpperLimit=DES.delta_e_max
  Gain : Gain  Gain=AP.Pitch.Kp
  Gain1 : Gain  Gain=AP.Pitch.Kd
  Sum : Sum  Inputs=|+-
  Sum1 : Sum  Inputs=|+-
  Sum2 : Sum  Inputs=++|
  delta_e : Outport
  wires:
  Gain/1 -> Sum1/1
  Sum/1 -> Gain/1
  Sum2/1 -> Elevator Saturation/1  "delta_e_unsat"
  theta_hat/1 -> Sum/2
  Gain1/1 -> Sum1/2
  Sum1/1 -> Sum2/2  "Ddelta_e"
  delta_e_trim/1 -> Sum2/1
  q_hat/1 -> Gain1/1
  Elevator Saturation/1 -> delta_e/1  "delta_e"
  pitch_cmd/1 -> Sum/1

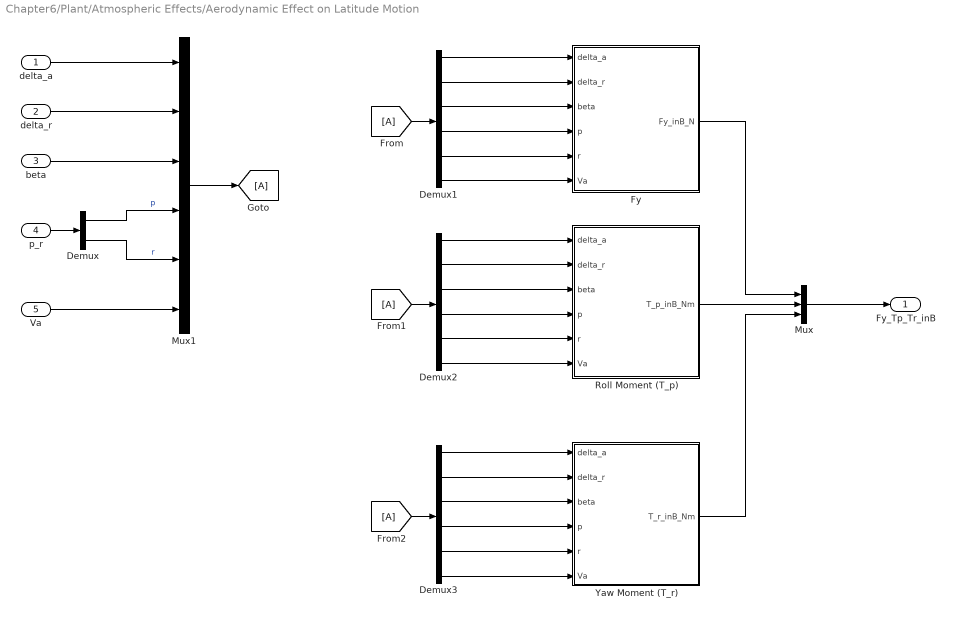
== system Chapter6/Plant/Atmospheric Effects/Aerodynamic Effect on Latitude Motion ==
  delta_a : Inport
  delta_r : Inport  Port=2
  beta : Inport  Port=3
  p_r : Inport  Port=4
  Va : Inport  Port=5
  Demux : Demux  Outputs=2
  Demux1 : Demux  Outputs=6
  Demux2 : Demux  Outputs=6
  Demux3 : Demux  Outputs=6
  From : From
  From1 : From
  From2 : From
  Fy : Subsystem
  Goto : Goto
  Mux : Mux  Inputs=3
  Mux1 : Mux  Inputs=6
  Roll Moment (T_p) : Subsystem
  Yaw Moment (T_r) : Subsystem
  Fy_Tp_Tr_inB : Outport
  wires:
  Mux/1 -> Fy_Tp_Tr_inB/1
  p_r/1 -> Demux/1
  Fy/1(Fy_inB_N) -> Mux/1
  Roll Moment (T_p)/1(T_p_inB_Nm) -> Mux/2
  Yaw Moment (T_r)/1(T_r_inB_Nm) -> Mux/3
  Demux1/1 -> Fy/1(delta_a)
  delta_a/1 -> Mux1/1
  delta_r/1 -> Mux1/2
  beta/1 -> Mux1/3
  Demux/1 -> Mux1/4  "p"
  Demux/2 -> Mux1/5  "r"
  Va/1 -> Mux1/6
  Mux1/1 -> Goto/1
  From/1 -> Demux1/1
  Demux1/2 -> Fy/2(delta_r)
  Demux1/3 -> Fy/3(beta)
  Demux1/4 -> Fy/4(p)
  Demux1/5 -> Fy/5(r)
  Demux1/6 -> Fy/6(Va)
  Demux2/4 -> Roll Moment (T_p)/4(p)
  Demux2/5 -> Roll Moment (T_p)/5(r)
  From1/1 -> Demux2/1
  Demux2/2 -> Roll Moment (T_p)/2(delta_r)
  Demux2/1 -> Roll Moment (T_p)/1(delta_a)
  Demux2/6 -> Roll Moment (T_p)/6(Va)
  Demux2/3 -> Roll Moment (T_p)/3(beta)
  Demux3/4 -> Yaw Moment (T_r)/4(p)
  Demux3/5 -> Yaw Moment (T_r)/5(r)
  From2/1 -> Demux3/1
  Demux3/2 -> Yaw Moment (T_r)/2(delta_r)
  Demux3/1 -> Yaw Moment (T_r)/1(delta_a)
  Demux3/6 -> Yaw Moment (T_r)/6(Va)
  Demux3/3 -> Yaw Moment (T_r)/3(beta)

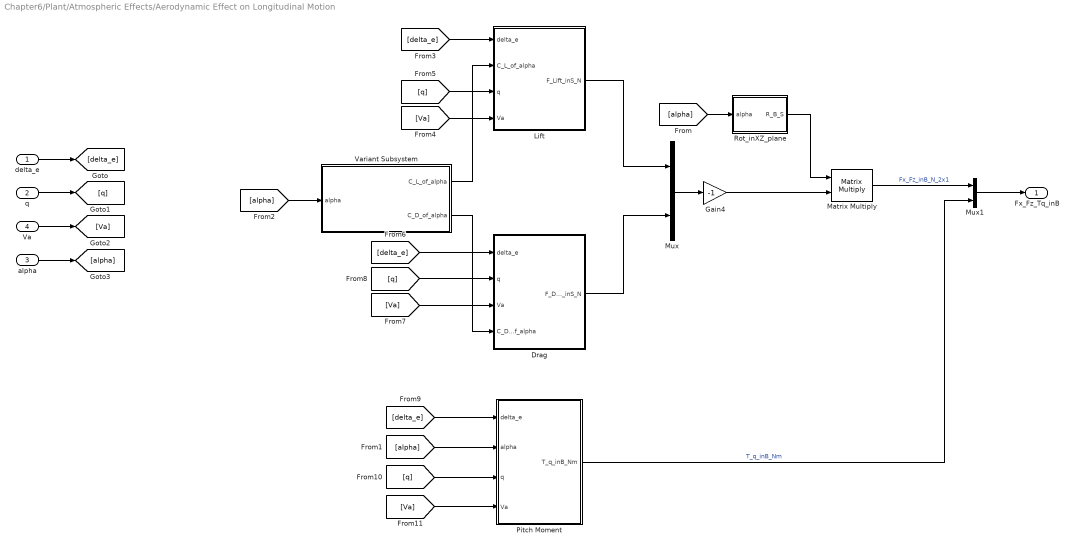
== system Chapter6/Plant/Atmospheric Effects/Aerodynamic Effect on Longitudinal Motion ==
  delta_e : Inport
  q : Inport  Port=2
  alpha : Inport  Port=3
  Va : Inport  Port=4
  Drag : Subsystem
  Gain4 : Gain  Gain=-1
  "Lift " : Subsystem
  Matrix Multiply : Product  Multiplication=Matrix(*)
  Mux : Mux  Inputs=2
  Mux1 : Mux  Inputs=2
  Pitch Moment : Subsystem
  Rot_inXZ_plane : MATLAB Function  TreatAsAtomicUnit=on
  Variant Subsystem : Subsystem  Variant=on
  Fx_Fz_Tq_inB : Outport
  wires:
  alpha/1 -> [alpha]
  [alpha] -> Rot_inXZ_plane/1(alpha)
  Mux/1 -> Gain4/1
  Rot_inXZ_plane/1(R_B_S) -> Matrix Multiply/1
  Gain4/1 -> Matrix Multiply/2
  Matrix Multiply/1 -> Mux1/1  "Fx_Fz_inB_N_2x1"
  Variant Subsystem/1(C_L_of_alpha) -> "Lift "/2(C_L_of_alpha)
  "Lift "/1(F_Lift_inS_N) -> Mux/1
  Variant Subsystem/2(C_D_of_alpha) -> Drag/4(C_D_of_alpha)
  Drag/1(F_Drag_inS_N) -> Mux/2
  Pitch Moment/1(T_q_inB_Nm) -> Mux1/2  "T_q_inB_Nm"
  Mux1/1 -> Fx_Fz_Tq_inB/1
  delta_e/1 -> [delta_e]
  Va/1 -> [Va]
  q/1 -> [q]
  [alpha] -> Variant Subsystem/1(alpha)
  [delta_e] -> "Lift "/1(delta_e)
  [Va] -> "Lift "/4(Va)
  [q] -> "Lift "/3(q)
  [delta_e] -> Drag/1(delta_e)
  [q] -> Drag/2(q)
  [Va] -> Drag/3(Va)
  [delta_e] -> Pitch Moment/1(delta_e)
  [q] -> Pitch Moment/3(q)
  [Va] -> Pitch Moment/4(Va)
  [alpha] -> Pitch Moment/2(alpha)

== system Chapter6/Plant/Subsystem1/Subsystem ==
  eta_I2B_rad_3x1 : Inport
  MATLAB Function : MATLAB Function  TreatAsAtomicUnit=on
  T_3x3 : Outport
  wires:
  eta_I2B_rad_3x1/1 -> MATLAB Function/1(u)
  MATLAB Function/1(y) -> T_3x3/1

== system Chapter6/Plant/Va-Alpha-Beta Extraction/norm2 ==
  Va_inB_m_s_3x1 : Inport
  Sqrt : Sqrt
  Square : Math  Operator=square
  Sum of Elements : Sum  Inputs=+
  Va : Outport
  wires:
  Va_inB_m_s_3x1/1 -> Square/1
  Square/1 -> Sum of Elements/1
  Sum of Elements/1 -> Sqrt/1
  Sqrt/1 -> Va/1

== system Chapter6/Autopilot/Lateral Autopilot/Course Hold Control Loop/Roll Hold Control Loop ==
  phi_cmd : Inport
  delta_a_trim : Inport  Port=2
  phi_hat : Inport  Port=3
  p_hat : Inport  Port=4
  Aileron Saturation : Saturate  UpperLimit=DES.delta_a_max  LowerLimit=-DES.delta_a_max
  Gain1 : Gain  Gain=AP.Roll.Kp
  Gain2 : Gain  Gain=-AP.Roll.Kd
  Gain3 : Gain  Gain=AP.Roll.Ki
  MATLAB Function : MATLAB Function  TreatAsAtomicUnit=on
  Roll Hold I Action : Integrator
  Sum : Sum  Inputs=|++
  Sum1 : Sum  Inputs=|+-
  Sum2 : Sum  Inputs=+++
  delta_a_sat : Outport
  wires:
  phi_cmd/1 -> Sum1/1
  Sum1/1 -> Gain1/1, Gain3/1
  Sum2/1 -> Sum/1  "Ddelta_a_unsat"
  phi_hat/1 -> Sum1/2
  p_hat/1 -> Gain2/1
  [u_unsat] -> MATLAB Function/1(u_unsat)
  [u_sat] -> MATLAB Function/2(u_sat)
  MATLAB Function/1(I) -> Roll Hold I Action/1
  Roll Hold I Action/1 -> Sum2/1
  Gain1/1 -> Sum2/2
  Gain2/1 -> Sum2/3
  delta_a_trim/1 -> Sum/2
  Sum/1 -> Aileron Saturation/1, [u_unsat]
  Aileron Saturation/1 -> delta_a_sat/1, [u_sat]
  Gain3/1 -> MATLAB Function/3(Ki_e)

== system Chapter6/Autopilot/Longitudinal Autopilot/Altitude Hold Control Outer Loop/WrapToPi ==
  In1 : Inport
  Constant : Constant  Value=pi
  Gain : Gain  Gain=2
  Mod : Math  Operator=mod
  Sum : Sum  Inputs=|++
  Sum1 : Sum  Inputs=|+-
  Out1 : Outport
  wires:
  In1/1 -> Sum/1
  Constant/1 -> Sum1/2, Gain/1, Sum/2
  Sum/1 -> Mod/1
  Gain/1 -> Mod/2
  Mod/1 -> Sum1/1
  Sum1/1 -> Out1/1

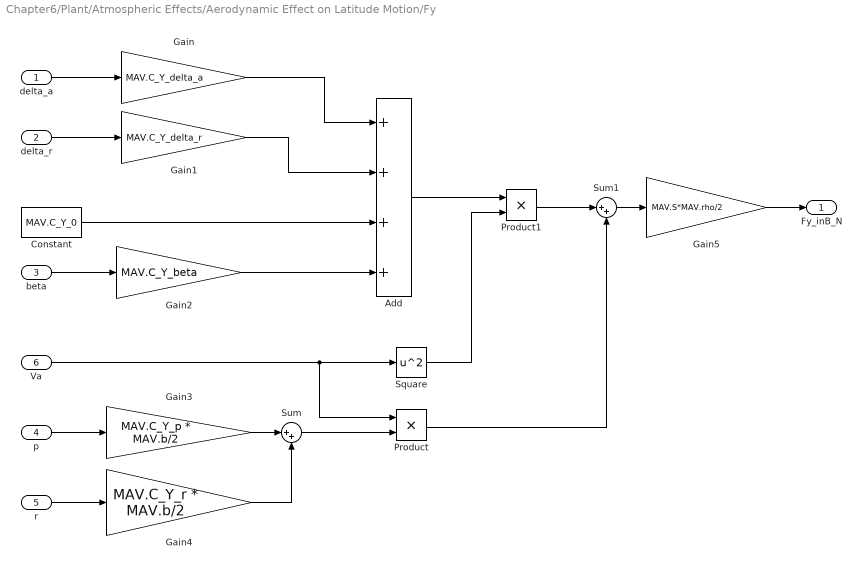
== system Chapter6/Plant/Atmospheric Effects/Aerodynamic Effect on Latitude Motion/Fy ==
  delta_a : Inport
  delta_r : Inport  Port=2
  beta : Inport  Port=3
  p : Inport  Port=4
  r : Inport  Port=5
  Va : Inport  Port=6
  Add : Sum  Inputs=++++
  Constant : Constant  Value=MAV.C_Y_0
  Gain : Gain  Gain=MAV.C_Y_delta_a
  Gain1 : Gain  Gain=MAV.C_Y_delta_r
  Gain2 : Gain  Gain=MAV.C_Y_beta
  Gain3 : Gain  Gain=MAV.C_Y_p * MAV.b/2
  Gain4 : Gain  Gain=MAV.C_Y_r * MAV.b/2
  Gain5 : Gain  Gain=MAV.S*MAV.rho/2
  Product : Product
  Product1 : Product
  Square : Math  Operator=square
  Sum : Sum  Inputs=|++
  Sum1 : Sum  Inputs=|++
  Fy_inB_N : Outport
  wires:
  delta_a/1 -> Gain/1
  delta_r/1 -> Gain1/1
  Constant/1 -> Add/3
  beta/1 -> Gain2/1
  Gain2/1 -> Add/4
  p/1 -> Gain3/1
  r/1 -> Gain4/1
  Gain3/1 -> Sum/1
  Gain4/1 -> Sum/2
  Gain/1 -> Add/1
  Gain1/1 -> Add/2
  Sum/1 -> Product/2
  Va/1 -> Square/1, Product/1
  Add/1 -> Product1/1
  Square/1 -> Product1/2
  Product1/1 -> Sum1/1
  Product/1 -> Sum1/2
  Sum1/1 -> Gain5/1
  Gain5/1 -> Fy_inB_N/1

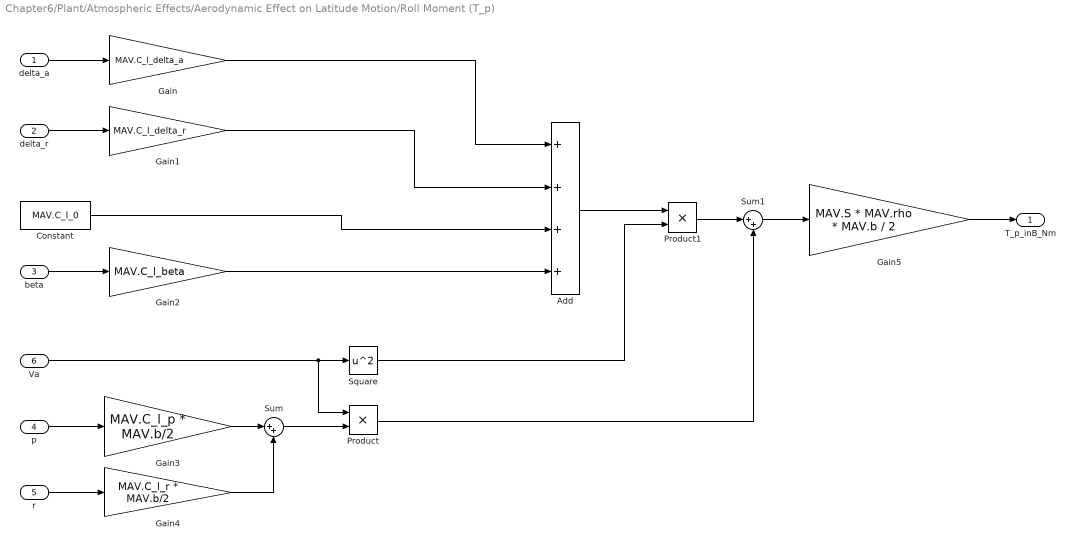
== system Chapter6/Plant/Atmospheric Effects/Aerodynamic Effect on Latitude Motion/Roll Moment (T_p) ==
  delta_a : Inport
  delta_r : Inport  Port=2
  beta : Inport  Port=3
  p : Inport  Port=4
  r : Inport  Port=5
  Va : Inport  Port=6
  Add : Sum  Inputs=++++
  Constant : Constant  Value=MAV.C_l_0
  Gain : Gain  Gain=MAV.C_l_delta_a
  Gain1 : Gain  Gain=MAV.C_l_delta_r
  Gain2 : Gain  Gain=MAV.C_l_beta
  Gain3 : Gain  Gain=MAV.C_l_p * MAV.b/2
  Gain4 : Gain  Gain=MAV.C_l_r * MAV.b/2
  Gain5 : Gain  Gain=MAV.S * MAV.rho * MAV.b / 2
  Product : Product
  Product1 : Product
  Square : Math  Operator=square
  Sum : Sum  Inputs=|++
  Sum1 : Sum  Inputs=|++
  T_p_inB_Nm : Outport
  wires:
  Gain1/1 -> Add/2
  Gain/1 -> Add/1
  Va/1 -> Square/1, Product/1
  Sum/1 -> Product/2
  Gain4/1 -> Sum/2
  Gain3/1 -> Sum/1
  r/1 -> Gain4/1
  p/1 -> Gain3/1
  Gain2/1 -> Add/4
  beta/1 -> Gain2/1
  Constant/1 -> Add/3
  delta_r/1 -> Gain1/1
  delta_a/1 -> Gain/1
  Add/1 -> Product1/1
  Square/1 -> Product1/2
  Product1/1 -> Sum1/1
  Product/1 -> Sum1/2
  Sum1/1 -> Gain5/1
  Gain5/1 -> T_p_inB_Nm/1

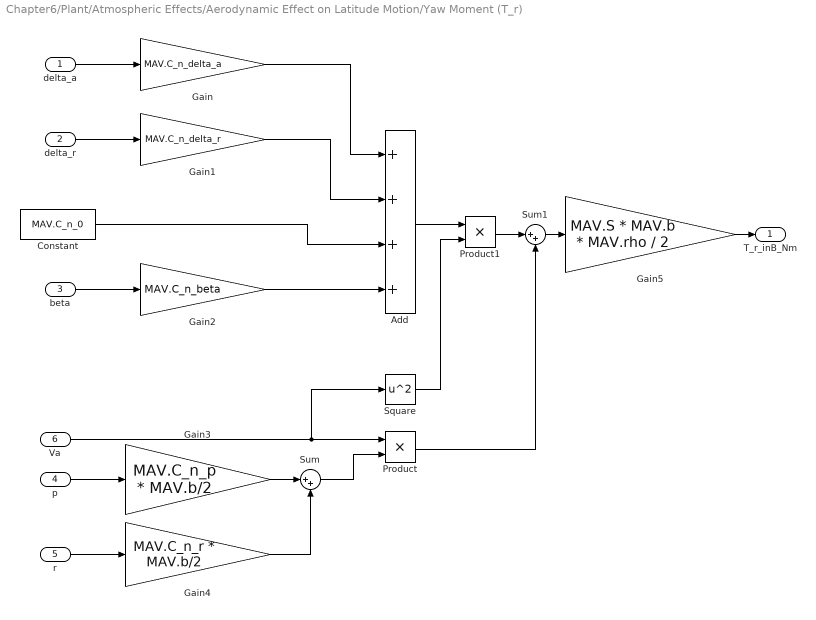
== system Chapter6/Plant/Atmospheric Effects/Aerodynamic Effect on Latitude Motion/Yaw Moment (T_r) ==
  delta_a : Inport
  delta_r : Inport  Port=2
  beta : Inport  Port=3
  p : Inport  Port=4
  r : Inport  Port=5
  Va : Inport  Port=6
  Add : Sum  Inputs=++++
  Constant : Constant  Value=MAV.C_n_0
  Gain : Gain  Gain=MAV.C_n_delta_a
  Gain1 : Gain  Gain=MAV.C_n_delta_r
  Gain2 : Gain  Gain=MAV.C_n_beta
  Gain3 : Gain  Gain=MAV.C_n_p * MAV.b/2
  Gain4 : Gain  Gain=MAV.C_n_r * MAV.b/2
  Gain5 : Gain  Gain=MAV.S * MAV.b * MAV.rho / 2
  Product : Product
  Product1 : Product
  Square : Math  Operator=square
  Sum : Sum  Inputs=|++
  Sum1 : Sum  Inputs=|++
  T_r_inB_Nm : Outport
  wires:
  Gain2/1 -> Add/4
  Constant/1 -> Add/3
  Gain1/1 -> Add/2
  delta_a/1 -> Gain/1
  p/1 -> Gain3/1
  Sum/1 -> Product/2
  Gain/1 -> Add/1
  r/1 -> Gain4/1
  Va/1 -> Square/1, Product/1
  Gain3/1 -> Sum/1
  delta_r/1 -> Gain1/1
  beta/1 -> Gain2/1
  Gain4/1 -> Sum/2
  Add/1 -> Product1/1
  Square/1 -> Product1/2
  Product1/1 -> Sum1/1
  Product/1 -> Sum1/2
  Sum1/1 -> Gain5/1
  Gain5/1 -> T_r_inB_Nm/1

== system Chapter6/Plant/Atmospheric Effects/Aerodynamic Effect on Longitudinal Motion/Drag ==
  delta_e : Inport
  q : Inport  Port=2
  Va : Inport  Port=3
  C_D_of_alpha : Inport  Port=4
  Gain : Gain  Gain=MAV.S * MAV.rho / 2
  Gain2 : Gain  Gain=MAV.C_D_delta_e
  Gain3 : Gain  Gain=MAV.C_D_q * MAV.c / 2
  Product : Product
  Product1 : Product
  Square : Math  Operator=square
  Sum : Sum  Inputs=|++
  Sum1 : Sum  Inputs=|++
  F_Drag_inS_N : Outport
  wires:
  Gain2/1 -> Sum/2
  delta_e/1 -> Gain2/1
  C_D_of_alpha/1 -> Sum/1
  q/1 -> Gain3/1
  Va/1 -> Square/1, Product/1
  Gain3/1 -> Product/2
  Sum/1 -> Product1/1
  Square/1 -> Product1/2
  Product1/1 -> Sum1/1
  Product/1 -> Sum1/2
  Sum1/1 -> Gain/1
  Gain/1 -> F_Drag_inS_N/1

== system Chapter6/Plant/Atmospheric Effects/Aerodynamic Effect on Longitudinal Motion/Lift  ==
  delta_e : Inport
  C_L_of_alpha : Inport  Port=2
  q : Inport  Port=3
  Va : Inport  Port=4
  Gain : Gain  Gain=MAV.C_L_delta_e
  Gain1 : Gain  Gain=MAV.C_L_q * MAV.c / 2
  Gain2 : Gain  Gain=MAV.S * MAV.rho / 2
  Product : Product
  Product1 : Product
  Square : Math  Operator=square
  Sum : Sum  Inputs=|++
  Sum1 : Sum  Inputs=|++
  F_Lift_inS_N : Outport
  wires:
  Gain/1 -> Sum/1
  C_L_of_alpha/1 -> Sum/2
  delta_e/1 -> Gain/1
  q/1 -> Gain1/1
  Gain1/1 -> Product/2
  Va/1 -> Product/1, Square/1
  Sum/1 -> Product1/1
  Square/1 -> Product1/2
  Product1/1 -> Sum1/1
  Product/1 -> Sum1/2
  Sum1/1 -> Gain2/1
  Gain2/1 -> F_Lift_inS_N/1

== system Chapter6/Plant/Atmospheric Effects/Aerodynamic Effect on Longitudinal Motion/Pitch Moment ==
  delta_e : Inport
  alpha : Inport  Port=2
  q : Inport  Port=3
  Va : Inport  Port=4
  Add1 : Sum  Inputs=+++
  Constant : Constant  Value=MAV.C_M_0
  Gain : Gain  Gain=MAV.S * MAV.rho * MAV.c / 2
  Gain1 : Gain  Gain=MAV.C_M_alpha
  Gain2 : Gain  Gain=MAV.C_M_delta_e
  Gain3 : Gain  Gain=MAV.C_M_q * MAV.c / 2
  Product : Product
  Product1 : Product
  Square : Math  Operator=square
  Sum : Sum  Inputs=|++
  T_q_inB_Nm : Outport
  wires:
  delta_e/1 -> Gain2/1
  Gain2/1 -> Add1/1
  alpha/1 -> Gain1/1
  Gain1/1 -> Add1/2
  Constant/1 -> Add1/3
  q/1 -> Gain3/1
  Gain3/1 -> Product/2
  Va/1 -> Product/1, Square/1
  Add1/1 -> Product1/1
  Square/1 -> Product1/2
  Product1/1 -> Sum/1
  Product/1 -> Sum/2
  Sum/1 -> Gain/1
  Gain/1 -> T_q_inB_Nm/1

== system Chapter6/Plant/Atmospheric Effects/Aerodynamic Effect on Longitudinal Motion/Variant Subsystem ==
  note: 1) Add Subsystem or Model blocks as valid variant choices.
      | 2) You cannot connect blocks at this level. At simulation, connectivity is automatically
      | determined, based on the active variant and port name matching.
  alpha : Inport
  Linear Lift Drag Effect of Alpha : Subsystem  VariantControl=LNG_MODEL == 1
  Nonlinear Lift Drag Effect of Alpha : Subsystem  VariantControl=LNG_MODEL == 2
  C_L_of_alpha : Outport
  C_D_of_alpha : Outport  Port=2

== system Chapter6/Plant/Atmospheric Effects/Aerodynamic Effect on Longitudinal Motion/Variant Subsystem/Linear Lift Drag Effect of Alpha ==
  alpha : Inport
  Constant : Constant  Value=MAV.C_L0_
  Constant1 : Constant  Value=MAV.C_D0_
  Gain : Gain  Gain=MAV.C_L_alpha
  Gain1 : Gain  Gain=MAV.C_D_alpha
  Sum : Sum  Inputs=++|
  Sum1 : Sum  Inputs=|++
  C_L_of_alpha : Outport
  C_D_of_alpha : Outport  Port=2
  wires:
  Gain/1 -> Sum/2
  Constant/1 -> Sum/1
  Sum/1 -> C_L_of_alpha/1
  alpha/1 -> Gain1/1, Gain/1
  Gain1/1 -> Sum1/1
  Constant1/1 -> Sum1/2
  Sum1/1 -> C_D_of_alpha/1

== system Chapter6/Plant/Atmospheric Effects/Aerodynamic Effect on Longitudinal Motion/Variant Subsystem/Nonlinear Lift Drag Effect of Alpha ==
  alpha : Inport
  Add : Sum
  Constant : Constant  Value=MAV.C_L0_
  Constant1 : Constant  Value=MAV.C_D_p
  Constant2 : Constant  Value=MAV.C_e * MAV.C_AR*pi
  Divide : Product  Inputs=*/
  Equation 4.10 : MATLAB Function  TreatAsAtomicUnit=on
  Equation 4.11 : Sum  Inputs=++|
  From : From
  Gain : Gain  Gain=MAV.C_L_alpha
  Goto : Goto
  Lift Flat Plate Coefficient Eq 4.8 : Subsystem
  Product : Product
  Product1 : Product
  Square : Math  Operator=square
  Sum : Sum  Inputs=++|
  C_L_of_alpha : Outport
  C_D_of_alpha : Outport  Port=2
  wires:
  Constant/1 -> Sum/1
  alpha/1 -> Lift Flat Plate Coefficient Eq 4.8/1(alpha), Equation 4.10/1(alpha), Gain/1
  Gain/1 -> Sum/2
  Sum/1 -> Goto/1, Product/1
  Equation 4.10/1(lambda1) -> Product/2
  Equation 4.10/2(lambda2) -> Product1/1
  Lift Flat Plate Coefficient Eq 4.8/1(C_L_flat_plate) -> Product1/2
  Product/1 -> Add/1
  Product1/1 -> Add/2
  Add/1 -> C_L_of_alpha/1
  From/1 -> Square/1
  Square/1 -> Divide/1
  Constant2/1 -> Divide/2
  Divide/1 -> Equation 4.11/2
  Constant1/1 -> Equation 4.11/1
  Equation 4.11/1 -> C_D_of_alpha/1

== system Chapter6/Plant/Atmospheric Effects/Aerodynamic Effect on Longitudinal Motion/Variant Subsystem/Nonlinear Lift Drag Effect of Alpha/Lift Flat Plate Coefficient Eq 4.8 ==
  alpha : Inport
  Cos : Trigonometry  Operator=cos
  Gain : Gain  Gain=2
  Product : Product  Inputs=3
  Sign : Signum
  Sin : Trigonometry
  Square : Math  Operator=square
  C_L_flat_plate : Outport
  wires:
  alpha/1 -> Cos/1, Sin/1, Sign/1
  Sin/1 -> Square/1
  Product/1 -> Gain/1
  Cos/1 -> Product/3
  Square/1 -> Product/2
  Sign/1 -> Product/1
  Gain/1 -> C_L_flat_plate/1

== matlab function Chapter6/Plant/Atmospheric Effects/Aerodynamic Effect on Longitudinal Motion/Rot_inXZ_plane ==
  data: alpha input; R_B_S output
function R_B_S = fcn(alpha)
    R_B_S = [-sin(alpha) cos(alpha);
             cos(alpha) sin(alpha)];
end

== matlab function Chapter6/Autopilot/Longitudinal Autopilot/MATLAB Function ==
  data: h_cmd input; zone output; h input; DES parameter
function zone = determineZone(h_cmd, h, DES)
    persistent current_zone;
    
    % --- SMART INITIALIZATION ---
    if isempty(current_zone)
        if h < DES.Altitude.Takeoff 
            current_zone = 0; % Take-off
        else
            current_zone = 2; % Hold
        end
    end
    
    err = h_cmd - h;
    enter_threshold = DES.Altitude.Threshold; 
    exit_threshold  = enter_threshold / 2; % Hysteresis
    
    % --- STATE MACHINE ---
    switch current_zone
        
        case 0 % --- TAKE-OFF ZONE ---
            if h > DES.Altitude.Takeoff
                current_zone = 1; % Climb Zone'a geç
            end

        case 1 % --- CLIMB ZONE ---
            if err < exit_threshold
                current_zone = 2; 
            end
            
        case 2 % --- HOLD ZONE --- 
            if err > enter_threshold
                current_zone = 1; % Climb
            elseif err < -enter_threshold
                current_zone = 3; % Descend
            end
            
        case 3 % --- DESCEND ZONE ---
            if err > -exit_threshold
                current_zone = 2; % Hold'a geç
            end
            
        otherwise
            current_zone = 2;
    end
    
    zone = current_zone;
end

== matlab function Chapter6/Plant/Atmospheric Effects/Aerodynamic Effect on Longitudinal Motion/Variant Subsystem/Nonlinear Lift Drag Effect of Alpha/Equation 4.10 ==
  data: alpha input; lambda1 output; MAV parameter; lambda2 output
function [lambda1, lambda2] = fcn(alpha, MAV)
% Equation 4.9 - 4.10    
exp_m = exp(-MAV.M * (alpha - MAV.alpha_0));
exp_p = exp(MAV.M * (alpha + MAV.alpha_0));
lambda2 = ( 1 + exp_m + exp_p) / ((1 + exp_m)*(1 + exp_p));
lambda1 = 1 - lambda2;
end

== matlab function Chapter6/Plant/Gravitational Force/R_B_I_c3 ==
  data: u input; y output
function y = fcn(u)
    y = zeros(3,1);
    y(1) = -sin(u(2));
    y(2) = cos(u(2)) * sin(u(1));
    y(3) = cos(u(2)) * cos(u(1));
end

== matlab function Chapter6/Plant/Subsystem1/MATLAB Function ==
  data: u input; y output
function y = fcn(u)
    y = wrapToPi(u);
